simulink model "force_position_step1"  (R2025b)
settings: Solver=VariableStepAuto  StartTime=0.0  StopTime=1.2  RelTol=1e-3
settings Model: Creator=HYB  LastModifiedBy=HYB

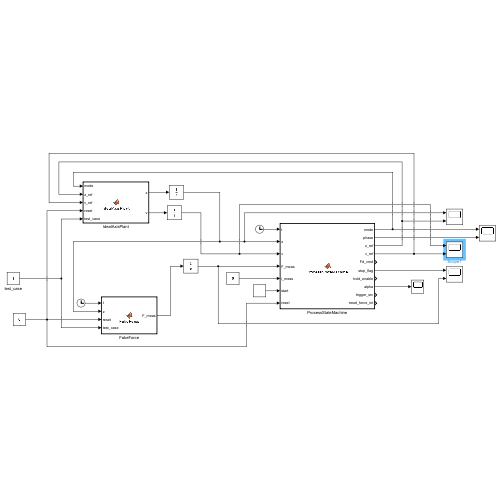
[thumbnail: Simulink's stored preview of the top-level diagram]
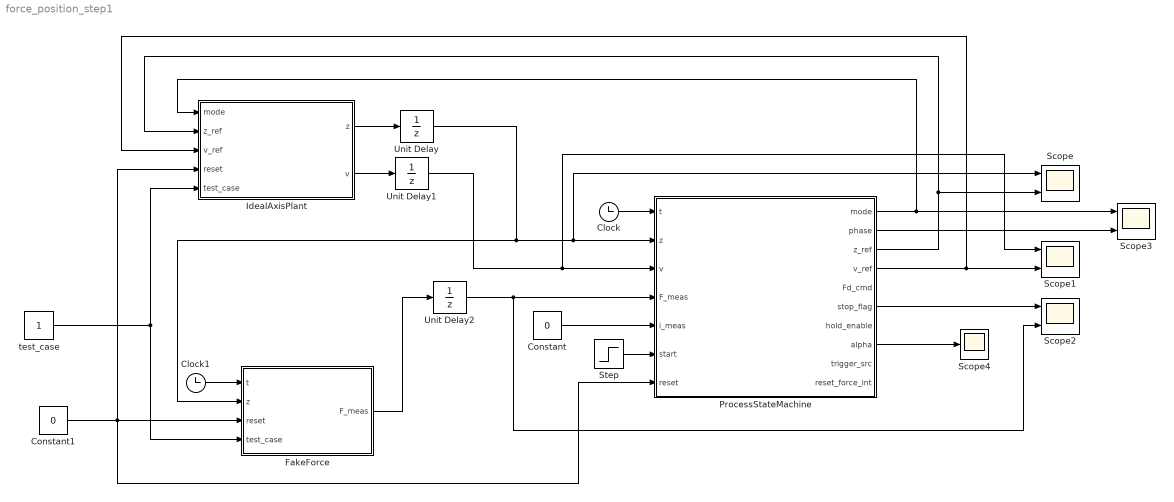
== system force_position_step1 ==
  Clock : Clock
  Clock1 : Clock
  Constant : Constant  Value=0
  Constant1 : Constant  Value=0
  FakeForce : MATLAB Function  TreatAsAtomicUnit=on
  IdealAxisPlant : MATLAB Function  TreatAsAtomicUnit=on
  ProcessStateMachine : MATLAB Function  TreatAsAtomicUnit=on
  Scope{,1..3} (4 alike) : Scope  NumInputPorts=2
      Scope settings: ActiveDisplayYMinimum=-1.8081940419150389  ActiveDisplayYMaximum=16.326241486595656
      Scope1 settings: ActiveDisplayYMinimum=-1.093190910866396  ActiveDisplayYMaximum=10.565960812431786
      Scope2 settings: ActiveDisplayYMinimum=-3.44979552873005  ActiveDisplayYMaximum=21.55020447126995  DataLoggingVariableName=ScopeData2
      Scope3 settings: ActiveDisplayYMinimum=-0.49999999999999989  ActiveDisplayYMaximum=4.5  DataLoggingVariableName=ScopeData3
  Scope4 : Scope
      settings: ActiveDisplayYMinimum=-0.12499999999999997  ActiveDisplayYMaximum=1.125  DataLoggingVariableName=ScopeData4
  Step : Step  Time=0.01  SampleTime=0
  Unit Delay : UnitDelay  SampleTime=0.001  HasFrameUpgradeWarning=on
  Unit Delay1 : UnitDelay  SampleTime=0.001  HasFrameUpgradeWarning=on
  Unit Delay2 : UnitDelay  SampleTime=0.001  HasFrameUpgradeWarning=on
  test_case : Constant
  wires:
  Clock/1 -> ProcessStateMachine/1(t)
  Step/1 -> ProcessStateMachine/6(start)
  Constant/1 -> ProcessStateMachine/5(i_meas)
  test_case/1 -> IdealAxisPlant/5(test_case), FakeForce/4(test_case)
  Constant1/1 -> FakeForce/3(reset), ProcessStateMachine/7(reset), IdealAxisPlant/4(reset)
  IdealAxisPlant/1(z) -> Unit Delay/1
  Unit Delay/1 -> FakeForce/2(z), Scope/1, ProcessStateMachine/2(z)
  IdealAxisPlant/2(v) -> Unit Delay1/1
  Unit Delay1/1 -> Scope1/1, ProcessStateMachine/3(v)
  FakeForce/1(F_meas) -> Unit Delay2/1
  Unit Delay2/1 -> Scope2/2, ProcessStateMachine/4(F_meas)
  ProcessStateMachine/3(z_ref) -> IdealAxisPlant/2(z_ref), Scope/2
  ProcessStateMachine/4(v_ref) -> Scope1/2, IdealAxisPlant/3(v_ref)
  ProcessStateMachine/1(mode) -> Scope3/1, IdealAxisPlant/1(mode)
  Clock1/1 -> FakeForce/1(t)
  ProcessStateMachine/6(stop_flag) -> Scope2/1
  ProcessStateMachine/2(phase) -> Scope3/2
  ProcessStateMachine/8(alpha) -> Scope4/1

== matlab function force_position_step1/IdealAxisPlant ==
  data: mode input; z output; z_ref input; v_ref input; reset input; v output; test_case input
function [z, v] = IdealAxisPlant(mode, z_ref, v_ref, reset, test_case)
%#codegen

% ============================================================
% 理想轴运动模型，仅用于测试状态机
% mode = 1：位置模式，快速逼近 z_ref
% mode = 2：速度模式，按 v_ref 运动
% mode = 3：力矩/保压模式，先假设位置保持
% mode = 9：错误停止
% ============================================================

Ts = 1e-3;          % 1 ms
z0 = 0.0;           % 初始位置 mm

v_pos_max = 50.0;   % 位置模式最大速度 mm/s
Kp_pos = 100.0;     % 理想位置跟踪增益

z_upper = 16.0;
z_lower = 0.0;

% 用于测试速度触发条件
z_obstacle = 14.5;

persistent z_k

if isempty(z_k)
    z_k = z0;
end

if reset
    z_k = z0;
end

v_cmd = 0.0;

if mode == 1
    % 位置模式：用简单比例控制逼近 z_ref
    err = z_ref - z_k;
    v_cmd = Kp_pos * err;
    
    if v_cmd > v_pos_max
        v_cmd = v_pos_max;
    elseif v_cmd < -v_pos_max
        v_cmd = -v_pos_max;
    end
    
    if abs(err) < 0.005
        z_k = z_ref;
        v_cmd = 0.0;
    end
    
elseif mode == 2
    % 速度模式
    v_cmd = v_ref;
    
    % test_case = 4 时，模拟碰到硬物后速度降为 0
    if test_case == 4 && z_k >= z_obstacle
        v_cmd = 0.0;
    end
    
elseif mode == 3
    % 力矩/保压模式：第一步测试中先假设保持当前位置
    v_cmd = 0.0;
    
elseif mode == 9
    % 安全停止
    v_cmd = 0.0;
    
else
    v_cmd = 0.0;
end

% 积分得到位置
z_k = z_k + Ts * v_cmd;

% 行程保护
if z_k > z_upper
    z_k = z_upper;
elseif z_k < z_lower
    z_k = z_lower;
end

z = z_k;
v = v_cmd;

== matlab function force_position_step1/ProcessStateMachine ==
  data: t input; mode output; z input; v input; F_meas input; i_meas input; start input; reset input; phase output; z_ref output; v_ref output; Fd_cmd output; stop_flag output; hold_enable output; alpha output; trigger_src output; reset_force_int output
function [mode, phase, z_ref, v_ref, Fd_cmd, stop_flag, hold_enable, alpha, trigger_src, reset_force_int] = ...
    ProcessStateMachine(t, z, v, F_meas, i_meas, start, reset)
%#codegen

% ============================================================
% 力位控制工艺流程状态机
% 阶段：
% 0 Ready
% 1 FastPosition: 位置模式快进到 13 mm
% 2 FirstVelocity: 第一速度到 14 mm
% 3 SearchVelocity: 第二速度搜索接触
% 4 ForceHold: 力矩/电流模式保压
% 5 ErrorStop: 超行程或异常停止
% ============================================================


%% ---------- 可调参数 ----------
z_fast_end = 13.0;     % mm
z_v1_end   = 14.0;     % mm
z_max      = 15.0;     % mm

pos_tol = 0.02;        % mm

v1_search = 5.0;       % mm/s
v2_search = 1.0;       % mm/s

F_th = 10.0;           % g
T_force_confirm = 0.002;   % s

v_stop_th = 0.05;          % mm/s
T_v_confirm = 0.005;       % s

% 第一版暂不启用电流判断，所以阈值给很大
i_stop_th = 1e9;
T_i_confirm = 0.003;       % s

Fd_set = 200.0;            % g
T_ramp_force = 0.010;      % s

%% ---------- 状态变量 ----------
persistent state t_enter tF_start tV_start tI_start prev_state

if isempty(state)
    state = int32(0);
    prev_state = int32(0);
    t_enter = 0.0;
    tF_start = -1.0;
    tV_start = -1.0;
    tI_start = -1.0;
end

if reset
    state = int32(0);
    prev_state = int32(0);
    t_enter = t;
    tF_start = -1.0;
    tV_start = -1.0;
    tI_start = -1.0;
end

%% ---------- 默认输出 ----------
mode = 0;
phase = double(state);
z_ref = z;
v_ref = 0.0;
Fd_cmd = Fd_set;
stop_flag = false;
hold_enable = false;
alpha = 0.0;
trigger_src = 0;       % 0 none, 1 force, 2 velocity, 3 current, 4 z_max
reset_force_int = false;

prev_state = state;

%% ---------- 启动逻辑 ----------
if state == 0
    mode = 0;
    phase = 0;
    z_ref = z;
    v_ref = 0.0;
    alpha = 0.0;
    
    if start
        state = int32(1);
        t_enter = t;
    end
end

%% ---------- 状态 1：位置快进 ----------
if state == 1
    mode = 1;          % 位置模式
    phase = 1;
    z_ref = z_fast_end;
    v_ref = 0.0;
    alpha = 0.0;
    
    if z >= z_fast_end - pos_tol
        state = int32(2);
        t_enter = t;
    end
end

%% ---------- 状态 2：第一速度 ----------
if state == 2
    mode = 2;          % 速度模式
    phase = 2;
    z_ref = z;
    v_ref = v1_search;
    alpha = 0.0;
    
    if z >= z_v1_end - pos_tol
        state = int32(3);
        t_enter = t;
        tF_start = -1.0;
        tV_start = -1.0;
        tI_start = -1.0;
    end
end

%% ---------- 状态 3：第二速度搜索 ----------
if state == 3
    mode = 2;          % 速度模式
    phase = 3;
    z_ref = z;
    v_ref = v2_search;
    alpha = 0.0;
    
    % --- 压力触发 ---
    if F_meas > F_th
        if tF_start < 0.0
            tF_start = t;
        end
    else
        tF_start = -1.0;
    end
    
    force_ok = false;
    if tF_start >= 0.0
        if (t - tF_start) >= T_force_confirm
            force_ok = true;
        end
    end
    
    % --- 速度触发，第一版作为备用 ---
    if abs(v) < v_stop_th
        if tV_start < 0.0
            tV_start = t;
        end
    else
        tV_start = -1.0;
    end
    
    velocity_ok = false;
    if tV_start >= 0.0
        if (t - tV_start) >= T_v_confirm
            velocity_ok = true;
        end
    end
    
    % --- 电流触发，第一版实际不会触发 ---
    if abs(i_meas) > i_stop_th
        if tI_start < 0.0
            tI_start = t;
        end
    else
        tI_start = -1.0;
    end
    
    current_ok = false;
    if tI_start >= 0.0
        if (t - tI_start) >= T_i_confirm
            current_ok = true;
        end
    end
    
    % --- 停止条件 ---
    if force_ok
        state = int32(4);
        t_enter = t;
        trigger_src = 1;
        stop_flag = true;
    elseif velocity_ok
        state = int32(4);
        t_enter = t;
        trigger_src = 2;
        stop_flag = true;
    elseif current_ok
        state = int32(4);
        t_enter = t;
        trigger_src = 3;
        stop_flag = true;
    elseif z >= z_max
        state = int32(5);
        t_enter = t;
        trigger_src = 4;
    end
end

%% ---------- 状态 4：力矩/电流模式保压 ----------
if state == 4
    mode = 3;          % 力矩/电流模式
    phase = 4;
    z_ref = z;
    v_ref = 0.0;
    Fd_cmd = Fd_set;
    stop_flag = true;
    hold_enable = true;
    
    % 目标力前馈平滑引入系数 alpha: 0 -> 1
    tau = (t - t_enter) / T_ramp_force;
    if tau < 0.0
        tau = 0.0;
    elseif tau > 1.0
        tau = 1.0;
    end
    
    % S型平滑
    alpha = 3.0*tau*tau - 2.0*tau*tau*tau;
end

%% ---------- 状态 5：安全停止 ----------
if state == 5
    mode = 9;
    phase = 5;
    z_ref = z;
    v_ref = 0.0;
    Fd_cmd = 0.0;
    stop_flag = true;
    hold_enable = false;
    alpha = 0.0;
end

%% ---------- 进入保压瞬间复位力控积分 ----------
if prev_state ~= int32(4) && state == int32(4)
    reset_force_int = true;
else
    reset_force_int = false;
end

phase = double(state);

== matlab function force_position_step1/FakeForce ==
  data: t input; z input; F_meas output; reset input; test_case input
function F_meas = FakeForce(t, z, reset, test_case)
%#codegen

% ============================================================
% 假力信号发生器，仅用于状态机测试
%
% test_case = 1：正常接触，z >= 14.5 mm 后持续产生力
% test_case = 2：始终无接触，测试最大行程保护
% test_case = 3：短暂误触发，测试持续时间确认逻辑
% test_case = 4：不产生力，配合 IdealAxisPlant 测试速度停止触发
% ============================================================

z_contact = 14.5;      % mm
F_contact = 20.0;      % g

persistent t_cross crossed

if isempty(t_cross)
    t_cross = -1.0;
    crossed = false;
end

if reset
    t_cross = -1.0;
    crossed = false;
end

F_meas = 0.0;

if test_case == 1
    % 正常接触：到达 14.5 mm 后持续有力
    if z >= z_contact
        F_meas = F_contact;
    else
        F_meas = 0.0;
    end
    
elseif test_case == 2
    % 无接触：始终为 0
    F_meas = 0.0;
    
elseif test_case == 3
    % 短暂误触发：只给 1 ms 左右的力脉冲
    if z >= z_contact && ~crossed
        crossed = true;
        t_cross = t;
    end
    
    if crossed
        if (t - t_cross) <= 0.001
            F_meas = F_contact;
        else
            F_meas = 0.0;
        end
    end
    
elseif test_case == 4
    % 不产生力，用于测试速度触发条件
    F_meas = 0.0;
    
else
    F_meas = 0.0;
end
